simulink model "commhdlQPSKTxRxLoopback"  (R2025b)
settings: Solver=FixedStepDiscrete  StartTime=0.0  StopTime=0.03  RelTol=1e-3
PostLoadFcn:
  | hScopeConfig = get_param([gcs '/Receiver/QPSK Rx/Frequency and Time Synchronizer/Symbol Synchronizer/No HDL/QPSK Receiver Eye Diagram'],'ScopeConfiguration');
  | 
  | hScopeConfig.OpenAtSimulationStart = false;
  | hScopeConfig.Visible = false;
  | SamplesPerSymbol = 4;
  | %UpsamplesRx = 1;
  | clear hScopeConfig
InitFcn:
  | % RxAlign decoder latency (flat_simfix): 41 = netlist value used for HDL; set
  | % rxAlignLat = 25 in the base workspace before a model-level simulation.
  | if ~exist('rxAlignLat','var'), rxAlignLat = uint16(41); end
  | commhdlQPSKTxRxModelInit;
  | % Rate bridge: ADRV9002/Jupiter radio runs at 15.36 MHz = 2x the 7.68 MHz
  | % (4 samples/symbol @ Rsym=1.92 MHz) the QPSK Rx requires. The deployed
  | % Receiver must downsample the ADC stream by 2. UpsamplesRx=1 fed the QPSK
  | % Rx 8 sps (2x-upsampled) and broke symbol sync / the loopback bit check.
  | UpsamplesRx = 1;   %% T8 RATE FIX: rail 15.36e6 == ADC bus rate,
  | %% no ingress decimation (was 2 when the rail sat on the 7.68e6 rung)
  | UpsamplesTx = 1;
  | clear simTimingOffset;
StopFcn:
  | if exist('simTimingOffset','var')
  |   disp('Simulation completed');
  |   %QPSKTxRxVerification;
  | end
undefined symbols (not defined in the file or in its folder): Add, Config, fsym, randsrc, RandStream, Rsym, rxAlignLat, Shift
libraries: hdlsllib x141, simulink x45, dspsigops x30, dsphdlfiltering2 x6, dsphdlsigops2 x4, dsphdlmathfun2 x4, commdigbbndpm3 x4, dspmlti4 x2, commchan3 x1, commrflib2 x1, commcnvcod2 x1
(part 5 of 9)

== system commhdlQPSKTxRxLoopback/Receiver/QPSK Rx/Frequency and Time Synchronizer/Preamble Detector/FIFO ==
  in : Inport
  push : Inport  Port=2
  pop : Inport  Port=3
  reset : Inport  Port=4
  Delay1 : Delay  DelayLength=1
  Pop Counter : hdlsllib/Sources/HDL Counter  CountType=Count limited  CountInit=0  CountStep=1  CountMax=fifoSize -1  CountFromType=Initial value  CountFrom=0  CountResetPort=on  CountLoadPort=off  CountEnbPort=on  CountDirPort=off  CountHitOutputPort=off  CountDataType=Unsigned  CountWordLen=nextpow2(fifoSize)  CountFracLen=0  CountSampTime=1
  Push Counter : hdlsllib/Sources/HDL Counter  CountType=Count limited  CountInit=0  CountStep=1  CountMax=fifoSize -1  CountFromType=Initial value  CountFrom=0  CountResetPort=on  CountLoadPort=off  CountEnbPort=on  CountDirPort=off  CountHitOutputPort=off  CountDataType=Unsigned  CountWordLen=nextpow2(fifoSize)  CountFracLen=0  CountSampTime=1
  Simple Dual Port RAM : hdlsllib/HDL RAMs/Simple Dual Port RAM  ram_size=nextpow2(fifoSize)
  Validate Input Push Pop : Subsystem
  out : Outport
  numEntries : Outport  Port=2
  validPop : Outport  Port=3
  wires:
  Delay1/1 -> Push Counter/1, Pop Counter/1
  in/1 -> Simple Dual Port RAM/1
  reset/1 -> Validate Input Push Pop/1(rst), Delay1/1
  Validate Input Push Pop/2(valid pop) -> Pop Counter/2, validPop/1
  Validate Input Push Pop/1(valid push) -> Push Counter/2, Simple Dual Port RAM/3
  pop/1 -> Validate Input Push Pop/3(pop)
  push/1 -> Validate Input Push Pop/2(push)
  Pop Counter/1 -> Simple Dual Port RAM/4
  Push Counter/1 -> Simple Dual Port RAM/2
  Simple Dual Port RAM/1 -> out/1
  Validate Input Push Pop/3(numEntries) -> numEntries/1

== system commhdlQPSKTxRxLoopback/Receiver/QPSK Rx/Frequency and Time Synchronizer/Preamble Detector/No HDL ==
  In1 : Inport
  In2 : Inport  Port=2
  Enable : EnablePort
  Correlation Time Scope : Scope  NumInputPorts=2
      settings: TimeUnits=Metric (based on Time Span)  Title=Time Plot of Preamble Detection  ActiveDisplayYMinimum=-0.38501295493915666  ActiveDisplayYMaximum=3.4651165944524109  YLabel=Amplitude
  Data Type Conversion : DataTypeConversion  OutDataTypeStr=double  SaturateOnIntegerOverflow=off  RndMeth=Floor
  Data Type Conversion1 : DataTypeConversion  OutDataTypeStr=double  SaturateOnIntegerOverflow=off  RndMeth=Floor
  To Workspace : ToWorkspace  VariableName=simPeakFind  SampleTime=-1
      settings: Save2DSignal=2-D array (concatenate along first dimension)
  wires:
  Data Type Conversion1/1 -> Correlation Time Scope/2  "Threshold"
  In2/1 -> Data Type Conversion1/1
  Data Type Conversion/1 -> To Workspace/1, Correlation Time Scope/1  "Correlation Value"
  In1/1 -> Data Type Conversion/1

== system commhdlQPSKTxRxLoopback/Receiver/QPSK Rx/Frequency and Time Synchronizer/Preamble Detector/Peak Search ==
  note: peak picker
  corr : Inport
  thresholdExceeded : Inport  Port=2
  validIn : Inport  Port=3
  Compare To Constant : simulink/Logic and Bit Operations/Compare To Constant  relop===  const=samplesPerFrame1x - 1  OutDataTypeStr=boolean
  Logical Operator : Logic  IconShape=distinctive  AllPortsSameDT=off  OutDataTypeStr=boolean
  Logical Operator4 : Logic  IconShape=distinctive  AllPortsSameDT=off  OutDataTypeStr=boolean
  Relational Operator : RelationalOperator  Operator=>  OutDataTypeStr=boolean  InputSameDT=off
  Terminator : Terminator
  Unit Delay Enabled Synchronous : hdlsllib/Discrete/Unit Delay Enabled Synchronous  InitialCondition=0.0  SampleTime=-1
  Unit Delay Enabled Synchronous1 : hdlsllib/Discrete/Unit Delay Enabled Synchronous  InitialCondition=0.0  SampleTime=-1
  Unit Delay Enabled Resettable Synchronous : hdlsllib/Discrete/Unit Delay Enabled Resettable Synchronous  InitialCondition=0.0  SampleTime=-1
  Unit Delay Enabled Resettable Synchronous1 : hdlsllib/Discrete/Unit Delay Enabled Resettable Synchronous  InitialCondition=0.0  SampleTime=-1
  timing Reference : hdlsllib/Sources/HDL Counter  CountType=Count limited  CountInit=0  CountStep=1  CountMax=samplesPerFrame1x - 1  CountFromType=Initial value  CountFrom=0  CountResetPort=off  CountLoadPort=off  CountEnbPort=on  CountDirPort=off  CountHitOutputPort=off  CountDataType=Unsigned  CountWordLen=nextpow2(samplesPerFrame1x - 1)  CountFracLen=0  CountSampTime=1
  timing Reference Long : hdlsllib/Sources/HDL Counter  CountType=Free running  CountInit=0  CountStep=1  CountMax=samplesPerFrame1x - 1  CountFromType=Initial value  CountFrom=0  CountResetPort=off  CountLoadPort=off  CountEnbPort=on  CountDirPort=off  CountHitOutputPort=off  CountDataType=Unsigned  CountWordLen=32  CountFracLen=0  CountSampTime=1
  timingOffset : Outport
  done : Outport  Port=2
  success : Outport  Port=3
  wires:
  validIn/1 -> Logical Operator/1, timing Reference/1, timing Reference Long/1
  timing Reference Long/1 -> Unit Delay Enabled Synchronous1/1
  timing Reference/1 -> Unit Delay Enabled Synchronous/1, Compare To Constant/1
  thresholdExceeded/1 -> Unit Delay Enabled Resettable Synchronous1/2, Unit Delay Enabled Resettable Synchronous1/1, Logical Operator4/2
  corr/1 -> Unit Delay Enabled Resettable Synchronous/1, Relational Operator/1
  Compare To Constant/1 -> Logical Operator/2
  Logical Operator/1 -> Unit Delay Enabled Resettable Synchronous1/3, done/1, Unit Delay Enabled Resettable Synchronous/3
  Relational Operator/1 -> Logical Operator4/1
  Unit Delay Enabled Resettable Synchronous/1 -> Relational Operator/2
  Unit Delay Enabled Resettable Synchronous1/1 -> success/1
  Logical Operator4/1 -> Unit Delay Enabled Synchronous/2, Unit Delay Enabled Synchronous1/2, Unit Delay Enabled Resettable Synchronous/2
  Unit Delay Enabled Synchronous/1 -> timingOffset/1
  Unit Delay Enabled Synchronous1/1 -> Terminator/1

== system commhdlQPSKTxRxLoopback/Receiver/QPSK Rx/Frequency and Time Synchronizer/Preamble Detector/Timing Adjust ==
  timingOffset : Inport
  timingOffsetValid : Inport  Port=2
  dataIn : Inport  Port=3
  validIn : Inport  Port=4
  Delay{,1..4} (5 alike) : Delay  DelayLength=1
  Logical Operator : Logic  AllPortsSameDT=off  OutDataTypeStr=boolean
  Logical Operator1 : Logic  Operator=NOT  AllPortsSameDT=off  OutDataTypeStr=boolean
  Logical Operator2 : Logic  Inputs=3  AllPortsSameDT=off  OutDataTypeStr=boolean
  No HDL : Subsystem
  Relational Operator : RelationalOperator  Operator===  OutDataTypeStr=boolean  InputSameDT=off
  State Register : hdlsllib/Discrete/Unit Delay Enabled Resettable Synchronous  InitialCondition=0.0  SampleTime=-1
  Unit Delay Enabled Synchronous3 : hdlsllib/Discrete/Unit Delay Enabled Synchronous  InitialCondition=0.0  SampleTime=-1
  timing Reference : hdlsllib/Sources/HDL Counter  CountType=Count limited  CountInit=0  CountStep=1  CountMax=searchSamples - 1  CountFromType=Initial value  CountFrom=0  CountResetPort=off  CountLoadPort=off  CountEnbPort=on  CountDirPort=off  CountHitOutputPort=off  CountDataType=Unsigned  CountWordLen=nextpow2(searchSamples - 1)  CountFracLen=0  CountSampTime=1
  dataOut : Outport
  validOut : Outport  Port=2
  SyncPulse : Outport  Port=3
  wires:
  Delay4/1 -> dataOut/1
  Delay3/1 -> validOut/1
  timingOffset/1 -> Unit Delay Enabled Synchronous3/1
  Unit Delay Enabled Synchronous3/1 -> Relational Operator/2
  Delay/1 -> SyncPulse/1
  validIn/1 -> timing Reference/1, Logical Operator2/1, No HDL/1(validIn), Delay3/1
  State Register/1 -> Logical Operator2/3, Delay1/1
  Logical Operator1/1 -> Logical Operator/2
  Relational Operator/1 -> Logical Operator2/2
  Logical Operator2/1 -> No HDL/3(syncPulse), Delay/1, Delay2/1
  Delay2/1 -> State Register/3
  Logical Operator/1 -> State Register/1, State Register/2, Unit Delay Enabled Synchronous3/2
  timing Reference/1 -> No HDL/2(timingOffset), Relational Operator/1
  timingOffsetValid/1 -> Logical Operator/1
  Delay1/1 -> Logical Operator1/1
  dataIn/1 -> Delay4/1

== system commhdlQPSKTxRxLoopback/Receiver/QPSK Rx/Frequency and Time Synchronizer/Symbol Synchronizer/Gardner TED ==
  data : Inport
  strobe : Inport  Port=2
  Constant : Constant  Value=0  OutDataTypeStr=Inherit: Inherit via back propagation  SampleTime=1/(Rsym*SamplesPerSymbol)
  Delay10 : Delay  DelayLength=4
  GTED : Subsystem
  Switch : Switch  Criteria=u2 ~= 0  InputSameDT=off
  e : Outport  VectorParamsAs1DForOutWhenUnconnected=off
  wires:
  Constant/1 -> Switch/3
  Switch/1 -> e/1
  strobe/1 -> Delay10/1
  data/1 -> GTED/1(In1)
  GTED/1(Out1) -> Switch/1
  Delay10/1 -> Switch/2

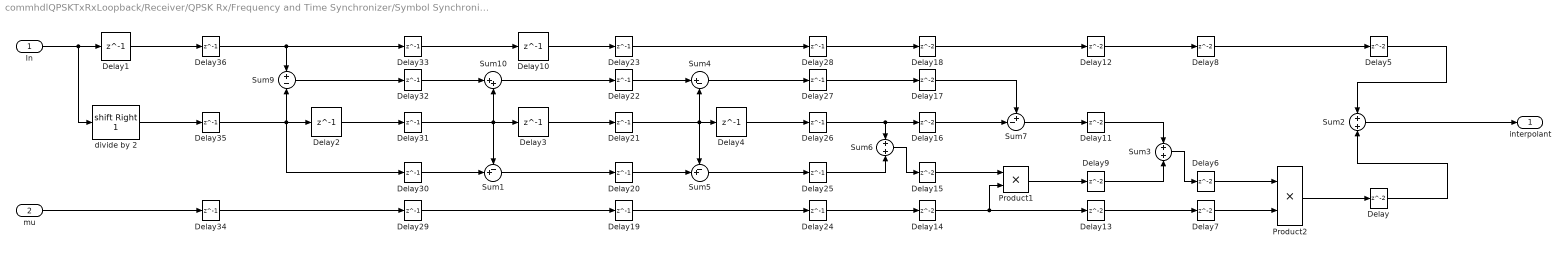
== system commhdlQPSKTxRxLoopback/Receiver/QPSK Rx/Frequency and Time Synchronizer/Symbol Synchronizer/Interpolation Filter ==
  In : Inport
  mu : Inport  Port=2
  Delay{,5..9,11..18} (14 alike) : Delay
  Delay{1..4,10} (5 alike) : Delay  DelayLength=1  InitialCondition=0
  Delay{19..36} (18 alike) : Delay  DelayLength=1
  Product1 : Product  OutDataTypeStr=fixdt(1,16,10)  RndMeth=Zero
  Product2 : Product  RndMeth=Zero  OutDataTypeStr=Inherit: Same as first input
  Sum1 : Sum  Inputs=-+|
  Sum10 : Sum  Inputs=|++
  Sum2 : Sum  Inputs=+|+
  Sum3 : Sum  Inputs=+|+  OutDataTypeStr=fixdt(1,16,10)
  Sum4 : Sum  Inputs=|+-
  Sum5 : Sum  Inputs=-+|
  Sum6 : Sum  Inputs=+|+  OutDataTypeStr=fixdt(1,16,11)  SaturateOnIntegerOverflow=on
  Sum7 : Sum  Inputs=+-|  OutDataTypeStr=fixdt(1,16,10)
  Sum9 : Sum  Inputs=+-
  divide by 2 : ArithShift  BitShiftNumber=1  BitShiftDirection=Right
  interpolant : Outport
  wires:
  Sum9/1 -> Delay32/1
  In/1 -> divide by 2/1, Delay1/1
  Sum2/1 -> interpolant/1
  Sum7/1 -> Delay11/1
  Product1/1 -> Delay9/1
  Product2/1 -> Delay/1
  Sum3/1 -> Delay6/1
  Sum1/1 -> Delay20/1
  Delay3/1 -> Delay21/1
  Sum10/1 -> Delay22/1
  Delay2/1 -> Delay31/1
  Delay1/1 -> Delay36/1
  divide by 2/1 -> Delay35/1
  Delay/1 -> Sum2/2
  Delay5/1 -> Sum2/1
  Delay6/1 -> Product2/1
  Delay7/1 -> Product2/2
  Delay8/1 -> Delay5/1
  Delay9/1 -> Sum3/2
  Delay11/1 -> Sum3/1
  Delay12/1 -> Delay8/1
  Delay13/1 -> Delay7/1
  Delay14/1 -> Delay13/1, Product1/2
  Delay15/1 -> Product1/1
  Delay16/1 -> Sum7/2
  Delay17/1 -> Sum7/1
  Delay18/1 -> Delay12/1
  mu/1 -> Delay34/1
  Sum5/1 -> Delay25/1
  Delay4/1 -> Delay26/1
  Sum4/1 -> Delay27/1
  Delay10/1 -> Delay23/1
  Delay24/1 -> Delay14/1
  Sum6/1 -> Delay15/1
  Delay26/1 -> Delay16/1, Sum6/1
  Delay27/1 -> Delay17/1
  Delay28/1 -> Delay18/1
  Delay25/1 -> Sum6/2
  Delay19/1 -> Delay24/1
  Delay20/1 -> Sum5/2
  Delay21/1 -> Sum4/2, Sum5/1, Delay4/1
  Delay22/1 -> Sum4/1
  Delay23/1 -> Delay28/1
  Delay29/1 -> Delay19/1
  Delay30/1 -> Sum1/2
  Delay31/1 -> Sum1/1, Sum10/2, Delay3/1
  Delay32/1 -> Sum10/1
  Delay33/1 -> Delay10/1
  Delay34/1 -> Delay29/1
  Delay35/1 -> Delay30/1, Delay2/1, Sum9/2
  Delay36/1 -> Delay33/1, Sum9/1

== system commhdlQPSKTxRxLoopback/Receiver/QPSK Rx/Frequency and Time Synchronizer/Symbol Synchronizer/Loop Filter ==
  note: Proportional-Plus-Integrator Loop Filter,
      | Infinite DC Response to guarantee convergence
  e : Inport
  Add : Sum
  Add2 : Sum  Inputs=|++  OutDataTypeStr=Inherit: Same as first input
  Data Type Conversion17 : DataTypeConversion  OutDataTypeStr=fixdt(1,11,10)  RndMeth=Floor
  Delay : Delay  DelayLength=1
  Delay1 : Delay  DelayLength=1  InitialCondition=0
  Delay2 : Delay  InitialCondition=0
  Delay3 : Delay  InitialCondition=0
  Delay4 : Delay  DelayLength=1  InitialCondition=0
  Delay5 : Delay  InitialCondition=0
  Delay6 : Delay  DelayLength=1
  IntegClamp : Saturate  UpperLimit=0.06  LowerLimit=-0.06
  K1 : Gain  Gain=fi(SSLoopFilterPropGain,1,24,24)  ParamDataTypeStr=Inherit: Inherit from 'Gain'  OutDataTypeStr=fixdt(1,30,23)
  K2 : Gain  Gain=fi(SSLoopFilterIntegGain,1,24,24)  ParamDataTypeStr=Inherit: Inherit from 'Gain'  OutDataTypeStr=fixdt(1,30,23)
  v : Outport
  wires:
  Delay/1 -> Add2/2
  Delay5/1 -> Delay6/1
  Delay3/1 -> Delay1/1
  e/1 -> Delay2/1
  Add/1 -> Data Type Conversion17/1
  Delay1/1 -> Add/1
  Delay4/1 -> Add/2
  Delay2/1 -> K1/1, K2/1
  Data Type Conversion17/1 -> v/1
  K2/1 -> Delay5/1
  K1/1 -> Delay3/1
  Delay6/1 -> Add2/1
  Add2/1 -> IntegClamp/1
  IntegClamp/1 -> Delay/1, Delay4/1

== system commhdlQPSKTxRxLoopback/Receiver/QPSK Rx/Frequency and Time Synchronizer/Symbol Synchronizer/No HDL ==
  data : Inport
  valid : Inport  Port=2
  Data Type Conversion : DataTypeConversion  OutDataTypeStr=double  SaturateOnIntegerOverflow=off  RndMeth=Floor
  No HDL : Subsystem
  QPSK Receiver Eye Diagram : EyeDiagramBlock  WindowPosition=[403.000000,370.000000,417.000000,506.000000,]  ScopeFrameLocation=window  SamplesPerSymbol=SamplesPerSymbol  SymbolsPerTrace=1  Title=RRC Matched Filtered Output  YLimits=[-1.1602,1.2629]
      settings: OpenAtSimulationStart=off
  Unit Delay Enabled Synchronous : hdlsllib/Discrete/Unit Delay Enabled Synchronous  InitialCondition=0.0  SampleTime=-1
  wires:
  data/1 -> No HDL/1(data), Unit Delay Enabled Synchronous/1
  Unit Delay Enabled Synchronous/1 -> Data Type Conversion/1
  valid/1 -> Unit Delay Enabled Synchronous/2, No HDL/Enable
  Data Type Conversion/1 -> QPSK Receiver Eye Diagram/1

== system commhdlQPSKTxRxLoopback/Receiver/QPSK Rx/Frequency and Time Synchronizer/Symbol Synchronizer/Rate Handle ==
  dataIn : Inport
  strobe : Inport  Port=2
  validIn : Inport  Port=3
  Compare To Constant : simulink/Logic and Bit Operations/Compare To Constant  relop===  const=0  OutDataTypeStr=boolean
  Constant : Constant  Value=false  SampleTime=-1
  FIFO : Subsystem  mask{fifoSize=32, pushFullDiag=Error, popEmptyDiag=Ignore}
      mask prompts: fifoSize "FIFO size:"; pushFullDiag "Push full FIFO:"; popEmptyDiag "Pop empty FIFO:"
      mask TypeOptions pushFullDiag: Ignore | Warning | Error
      mask TypeOptions popEmptyDiag: Ignore | Warning | Error
  HDL Counter : hdlsllib/Sources/HDL Counter  CountType=Count limited  CountInit=0  CountStep=1  CountMax=SamplesPerSymbol - 1  CountFromType=Initial value  CountFrom=0  CountResetPort=off  CountLoadPort=off  CountEnbPort=on  CountDirPort=off  CountHitOutputPort=off  CountDataType=Unsigned  CountWordLen=max(1, nextpow2(SamplesPerSymbol - 1))  CountFracLen=0  CountSampTime=1
  Logical Operator : Logic  AllPortsSameDT=off  OutDataTypeStr=boolean
  Terminator : Terminator
  dataOut : Outport
  validOut : Outport  Port=2
  wires:
  strobe/1 -> FIFO/2(push)
  dataIn/1 -> FIFO/1(in)
  validIn/1 -> Logical Operator/1, HDL Counter/1
  HDL Counter/1 -> Compare To Constant/1
  Compare To Constant/1 -> Logical Operator/2
  Logical Operator/1 -> FIFO/3(pop)
  FIFO/1(out) -> dataOut/1
  FIFO/3(validPop) -> validOut/1
  FIFO/2(numEntries) -> Terminator/1
  Constant/1 -> FIFO/4(reset)

== system commhdlQPSKTxRxLoopback/Transmitter/QPSK Tx/Bit Packetizer/Data Bits FIFO/No HDL ==
  push : Inport
  pop : Inport  Port=2
  MATLAB Function : MATLAB Function  TreatAsAtomicUnit=on
  No HDL : Subsystem
  wires:
  push/1 -> MATLAB Function/1(wr), No HDL/1(push)
  pop/1 -> MATLAB Function/2(rd), No HDL/5(pop)
  MATLAB Function/2(ncount) -> No HDL/3(ncount)
  MATLAB Function/1(full) -> No HDL/2(full)
  MATLAB Function/3(empty) -> No HDL/4(empty)

== system commhdlQPSKTxRxLoopback/Transmitter/QPSK Tx/Bit Packetizer/Preamble Bits Generator/Preamble Bits Store ==
  note: The Preamble is padded with zeros in the LUT such that
      | the length is the 2^nextpow2(length(Preamble)) for
      | efficient resource mapping to RAM
  actualPreamble : Inport
  sampleCount : Inport  Port=2
  Constant : Constant  OutDataTypeStr=boolean  SampleTime=1/(Rsym*SamplesPerSymbol)
  Extract Bits : simulink/Logic and Bit Operations/Extract Bits  bitsToExtract=Range of bits  numBits=8  bitIdxRange=[0 nextpow2(length(Preamble))-1]  outScalingMode=Treat bit field as an integer
  Preamble : LookupNDDirect  NumberOfTableDimensions=1  Table=[Preamble;false(32-length(Preamble),1)]  DiagnosticForOutOfRangeInput=Error
  Switch : Switch  Criteria=u2 ~= 0  Threshold=1  SaturateOnIntegerOverflow=off  InputSameDT=off
  preamble : Outport
  wires:
  Switch/1 -> preamble/1
  Constant/1 -> Switch/3
  Extract Bits/1 -> Preamble/1
  Preamble/1 -> Switch/1
  sampleCount/1 -> Extract Bits/1
  actualPreamble/1 -> Switch/2

== system commhdlQPSKTxRxLoopback/TxRxComposite/Receiver/QPSK Rx/Automatic Gain Control/Error Detector ==
  dataIn : Inport
  Add1 : Sum  Inputs=+-
  Conj : Math  Operator=conj
  Data Type Duplicate : DataTypeDuplicate
  Delay{,1..3} (4 alike) : Delay
  Product : Product
  Ref : Constant  Value=Ref  OutDataTypeStr=Inherit: Inherit via back propagation  SampleTime=-1
  err : Outport
  wires:
  Add1/1 -> Delay3/1
  Delay2/1 -> Add1/2
  Product/1 -> Delay2/1
  Delay/1 -> Product/2
  Delay3/1 -> err/1
  Delay1/1 -> Product/1
  Conj/1 -> Delay/1
  dataIn/1 -> Conj/1, Data Type Duplicate/2, Delay1/1
  Ref/1 -> Data Type Duplicate/1, Add1/1

== system commhdlQPSKTxRxLoopback/TxRxComposite/Receiver/QPSK Rx/Automatic Gain Control/Loop Filter ==
  note: Fixed point precision loss warnings
      | are supressed in Mask Init Callback
  err : Inport
  agc_loop_gain : Inport  Port=2  OutDataTypeStr=uint32  SampleTime=1/(Rsym*SamplesPerSymbol)
  Add : Sum  Inputs=|++  OutDataTypeStr=Inherit: Same as first input
  Delay1 : Delay  DelayLength=1
  Delay2 : Delay
  Delay3 : Delay
  Gain1 : Gain  Gain=LFG  OutDataTypeStr=fixdt(1,34,28)
      mask init:
      | Simulink.suppressDiagnostic(gcb, 'SimulinkFixedPoint:util:fxpParameterPrecisionLoss');
  LGMux_agc_loop_gain : MATLAB Function  TreatAsAtomicUnit=on
  LGProd_agc_loop_gain : Product  OutDataTypeStr=fixdt(1,34,28)
  LGSw_agc_loop_gain : Switch  Criteria=u2 ~= 0  OutDataTypeStr=fixdt(1,34,28)
  gain : Outport
  wires:
  LGSw_agc_loop_gain/1 -> Delay2/1
  LGProd_agc_loop_gain/1 -> LGSw_agc_loop_gain/1
  Delay1/1 -> gain/1, Add/2
  Delay3/1 -> LGProd_agc_loop_gain/1, Gain1/1
  Gain1/1 -> LGSw_agc_loop_gain/3
  LGMux_agc_loop_gain/2(nz) -> LGSw_agc_loop_gain/2
  err/1 -> Delay3/1
  Add/1 -> Delay1/1
  Delay2/1 -> Add/1
  LGMux_agc_loop_gain/1(coeff) -> LGProd_agc_loop_gain/2
  agc_loop_gain/1 -> LGMux_agc_loop_gain/1(axi)

== system commhdlQPSKTxRxLoopback/TxRxComposite/Receiver/QPSK Rx/FEC Decoder Wrapper/VitGate ==
  pairIn : Inport
  rstIn : Inport  Port=2
  Enable : EnablePort
  Viterbi : commcnvcod2/Viterbi Decoder  trellis=poly2trellis(5, [35 23])  isPunctured=off  punctureVector=[1; 1; 0; 1; 0; 1]  erasures=off  dectype=Hard decision  nsdecb=4  runSigValErrCheck=off  tbdepth=25  opmode=Continuous  reset=on  delayedResetAction=on  smWordLength=16  outDataType=boolean
  decOut : Outport
  wires:
  Viterbi/1 -> decOut/1
  rstIn/1 -> Viterbi/2
  pairIn/1 -> Viterbi/1

== system commhdlQPSKTxRxLoopback/TxRxComposite/Receiver/QPSK Rx/Frequency and Time Synchronizer/Carrier Synchronizer ==
  dataIn : Inport
  internalRst : Inport  Port=2
  validIn : Inport  Port=3
  manualRst : Inport  Port=4
  cs_prop_gain : Inport  Port=5  OutDataTypeStr=uint32  SampleTime=1/(Rsym*SamplesPerSymbol)
  cs_integ_gain : Inport  Port=6  OutDataTypeStr=uint32  SampleTime=1/(Rsym*SamplesPerSymbol)
  Data Type Conversion2 : DataTypeConversion  OutDataTypeStr=fixdt(1,16,14)  SaturateOnIntegerOverflow=off  RndMeth=Floor
  Delay{,2,5,7,11} (5 alike) : Delay  DelayLength=1
  Delay{1,10,14..15} (4 alike) : Delay  DelayLength=6
  Delay{3..4,6,8..9,12..13} (7 alike) : Delay
  Direct Digital Synthesis : Subsystem
  Logical Operator : Logic  AllPortsSameDT=off  OutDataTypeStr=boolean
  Loop Filter : Subsystem
  Math Function : Math  Operator=conj  SignedPower=on  RndMeth=Zero
  Phase Error Detector : Subsystem
  Product : Product
  dataOut : Outport
  validOut : Outport  Port=2
  wires:
  Delay5/1 -> dataOut/1
  Delay/1 -> Phase Error Detector/1(dataIn)
  Delay1/1 -> Loop Filter/2(validIn)
  Math Function/1 -> Delay3/1
  Data Type Conversion2/1 -> Delay5/1, Delay/1
  Loop Filter/3(rst) -> Logical Operator/2
  Loop Filter/2(valid) -> Direct Digital Synthesis/2(validIn)
  Delay3/1 -> Product/2
  Loop Filter/1(v) -> Direct Digital Synthesis/3(phaseInc)
  cs_integ_gain/1 -> Loop Filter/6(cs_integ_gain)
  cs_prop_gain/1 -> Loop Filter/5(cs_prop_gain)
  Delay12/1 -> Delay11/1
  internalRst/1 -> Delay13/1
  Delay2/1 -> Delay1/1
  Delay13/1 -> Delay12/1
  manualRst/1 -> Loop Filter/4(externalRst), Logical Operator/1
  Delay14/1 -> Delay9/1
  Delay4/1 -> Product/1
  Delay15/1 -> Loop Filter/3(internalRst)
  Delay9/1 -> Delay8/1
  Logical Operator/1 -> Direct Digital Synthesis/1(rst)
  validIn/1 -> Delay14/1
  Product/1 -> Delay6/1
  Delay8/1 -> Delay7/1, Delay2/1
  dataIn/1 -> Delay10/1
  Direct Digital Synthesis/1(expOut) -> Math Function/1
  Delay7/1 -> validOut/1
  Delay6/1 -> Data Type Conversion2/1
  Delay11/1 -> Delay15/1
  Delay10/1 -> Delay4/1
  Phase Error Detector/1(PhaseError) -> Loop Filter/1(e)

== system commhdlQPSKTxRxLoopback/TxRxComposite/Receiver/QPSK Rx/Frequency and Time Synchronizer/Coarse Frequency Compensator ==
  dataIn : Inport
  validIn : Inport  Port=2
  cfo_threshold : Inport  Port=3  OutDataTypeStr=uint32  SampleTime=1/(Rsym*SamplesPerSymbol)
  CFO step change detector : Subsystem
  Coarse Frequency Estimator : Subsystem
  Data Type Conversion2 : DataTypeConversion  OutDataTypeStr=fixdt(1,16,12)  SaturateOnIntegerOverflow=off  RndMeth=Floor
  Data Type Conversion3 : DataTypeConversion  OutDataTypeStr=fixdt(1,21,21)  SaturateOnIntegerOverflow=off  RndMeth=Floor
  Data Type Conversion4 : DataTypeConversion  OutDataTypeStr=fixdt(1,21,0)  ConvertRealWorld=Stored Integer (SI)  SaturateOnIntegerOverflow=off  RndMeth=Floor
  Delay1 : Delay  DelayLength=9
  Delay{11..17} (7 alike) : Delay
  Delay2 : Delay  DelayLength=9
  Delay3 : Delay  DelayLength=6
  Delay4 : Delay  DelayLength=6
  Delay5 : Delay  DelayLength=1
  Delay6 : Delay  DelayLength=1
  Delay7 : Delay  DelayLength=12
  Delay8 : Delay  DelayLength=12
  Gain : Gain  Gain=1/4  ParamDataTypeStr=fixdt(0,2,2)  OutDataTypeStr=Inherit: Same as input
  Math Function : Math  Operator=conj
  NCO : dsphdlsigops2/NCO  PhaseIncrementSource=Input port  PhaseIncrement=100  PhaseOffsetSource=Property  PhaseOffset=0  DitherSource=None  NumDitherBits=4  SamplesPerFrame=1  LUTCompress=off  ResetAction=off  Waveform=Complex exponential  PhasePort=off  SimulateUsing=Code generation  AccumulatorWL=21  PhaseQuantization=on  NumQuantizerAccumulatorBits=14  OutputDataType=Binary point scaling  OutputWL=16  OutputFL=14
  Product1 : Product  OutDataTypeStr=Inherit: Same as first input
  Raise Power to 4 : Subsystem
  Terminator : Terminator
  dataOut : Outport
  rstCS : Outport  Port=2
  validOut : Outport  Port=3
  normalizedFreqEst : Outport  Port=4
  wires:
  Delay8/1 -> Delay4/1, NCO/2
  Raise Power to 4/2(validOut) -> Coarse Frequency Estimator/2(validIn)
  Coarse Frequency Estimator/1(normFreqEst) -> Gain/1
  Delay2/1 -> Delay8/1
  cfo_threshold/1 -> CFO step change detector/2(cfo_threshold)
  Delay16/1 -> Delay17/1
  Delay6/1 -> Raise Power to 4/2(validIn), Delay2/1
  Delay3/1 -> Delay11/1
  Data Type Conversion2/1 -> Raise Power to 4/1(dataIn)
  Delay5/1 -> Data Type Conversion2/1, Delay1/1
  Raise Power to 4/1(dataOut) -> Coarse Frequency Estimator/1(dataIn)
  Delay7/1 -> Delay3/1
  Data Type Conversion4/1 -> NCO/1
  Delay1/1 -> Delay7/1
  Delay13/1 -> dataOut/1
  Product1/1 -> Delay13/1
  validIn/1 -> Delay6/1
  dataIn/1 -> Delay5/1
  Gain/1 -> Data Type Conversion3/1
  Delay4/1 -> Delay14/1
  Delay15/1 -> validOut/1
  Data Type Conversion3/1 -> normalizedFreqEst/1, CFO step change detector/1(In1), Data Type Conversion4/1
  CFO step change detector/1(Out1) -> Delay16/1
  NCO/1 -> Math Function/1
  NCO/2 -> Terminator/1
  Math Function/1 -> Delay12/1
  Delay17/1 -> rstCS/1
  Delay11/1 -> Product1/1
  Delay14/1 -> Delay15/1
  Delay12/1 -> Product1/2

== system commhdlQPSKTxRxLoopback/TxRxComposite/Receiver/QPSK Rx/Frequency and Time Synchronizer/No HDL ==
  In1 : Inport
  In2 : Inport  Port=2
  In3 : Inport  Port=3
  In4 : Inport  Port=4
  Data Type Conversion : DataTypeConversion  OutDataTypeStr=double  SaturateOnIntegerOverflow=off  RndMeth=Floor
  Data Type Conversion1 : DataTypeConversion  OutDataTypeStr=double  SaturateOnIntegerOverflow=off  RndMeth=Floor
  Subsystem : Subsystem
  Unit Delay Enabled Synchronous : hdlsllib/Discrete/Unit Delay Enabled Synchronous  InitialCondition=0.0  SampleTime=-1
  Unit Delay Enabled Synchronous1 : hdlsllib/Discrete/Unit Delay Enabled Synchronous  InitialCondition=0.0  SampleTime=-1
  wires:
  Data Type Conversion/1 -> Unit Delay Enabled Synchronous1/1, Subsystem/1(In1)
  In4/1 -> Unit Delay Enabled Synchronous1/2, Subsystem/Enable
  In2/1 -> Unit Delay Enabled Synchronous/2
  Data Type Conversion1/1 -> Unit Delay Enabled Synchronous/1
  In3/1 -> Data Type Conversion/1
  In1/1 -> Data Type Conversion1/1

== system commhdlQPSKTxRxLoopback/TxRxComposite/Receiver/QPSK Rx/Frequency and Time Synchronizer/Packet Controller ==
  dataIn : Inport
  syncPulse : Inport  Port=2
  validIn : Inport  Port=3
  Delay : Delay  DelayLength=4
  Delay1 : Delay  DelayLength=4
  Delay2 : Delay  DelayLength=4
  End Generator : Subsystem
  Logical Operator : Logic  IconShape=distinctive  AllPortsSameDT=off  OutDataTypeStr=boolean
  MATLAB Function : MATLAB Function  TreatAsAtomicUnit=on
  Time Scope End Generator : Scope  Commented=on  NumInputPorts=2
      settings: SampleTime=1  ActiveDisplayYMinimum=-0.048155737704917989  ActiveDisplayYMaximum=1.0464480874316939  YLabel=Amplitude  DataLoggingVariableName=ScopeData2
  sample discard controller : MATLAB Function  TreatAsAtomicUnit=on
  dataOut : Outport
  startOut : Outport  Port=2
  endOut : Outport  Port=3
  validOut : Outport  Port=4
  wires:
  sample discard controller/4(validOut) -> validOut/1
  Delay/1 -> sample discard controller/1(dataIn)
  sample discard controller/2(startOut) -> startOut/1
  End Generator/1(endOut) -> sample discard controller/4(endIn), Time Scope End Generator/1
  Logical Operator/1 -> Delay2/1, End Generator/2(rst), Time Scope End Generator/2
  Delay1/1 -> End Generator/1(validIn), sample discard controller/2(validIn)
  dataIn/1 -> Delay/1
  sample discard controller/1(dataOut) -> dataOut/1
  MATLAB Function/1(out) -> Logical Operator/2
  sample discard controller/3(endOut) -> endOut/1
  syncPulse/1 -> MATLAB Function/2(syncPulse)
  Delay2/1 -> sample discard controller/3(startIn)
  validIn/1 -> MATLAB Function/1(valid), Delay1/1, Logical Operator/1

== system commhdlQPSKTxRxLoopback/TxRxComposite/Receiver/QPSK Rx/Frequency and Time Synchronizer/Phase Ambiguity Estimation and Correction ==
  dataIn : Inport
  syncPulseIn : Inport  Port=2
  validIn : Inport  Port=3
  Average Estimates : Subsystem
  Delay : Delay  DelayLength=32
  Delay1 : Delay  DelayLength=32
  Delay10 : Delay  DelayLength=15 + 7
  Delay11 : Delay  DelayLength=5
  Delay12 : Delay  DelayLength=5
  Delay13 : Delay  DelayLength=5
  Delay2 : Delay  DelayLength=32
  Delay3 : Delay  DelayLength=8
  Delay4 : Delay  DelayLength=8
  Delay5 : Delay  DelayLength=8
  Delay6 : Delay  DelayLength=1
  Delay7 : Delay  DelayLength=1
  Delay8 : Delay  DelayLength=1
  Delay9 : Delay  DelayLength=10
  EstDataLookback : Delay  DelayLength=6
  EstVldLookback : Delay  DelayLength=6
  Phase Ambiguity Corrector : Subsystem
  Phase Ambiguity Estimator : Subsystem
  dataOut : Outport
  syncPulseOut : Outport  Port=2
  validOut : Outport  Port=3
  wires:
  Delay9/1 -> syncPulseOut/1
  Phase Ambiguity Corrector/2(validOut) -> validOut/1
  Phase Ambiguity Corrector/1(dataOut) -> dataOut/1
  Delay6/1 -> Delay10/1
  Average Estimates/1(avgEst) -> Phase Ambiguity Corrector/2(estimate)
  Delay8/1 -> Phase Ambiguity Corrector/1(dataIn)
  Delay3/1 -> Delay1/1
  Delay7/1 -> Phase Ambiguity Corrector/3(validIn)
  Delay/1 -> EstDataLookback/1, Delay13/1
  Delay1/1 -> Delay11/1
  Phase Ambiguity Estimator/3(validOut) -> Average Estimates/3(validIn)
  validIn/1 -> Delay4/1
  Delay4/1 -> Delay2/1
  Delay2/1 -> EstVldLookback/1, Delay12/1
  syncPulseIn/1 -> Phase Ambiguity Estimator/2(syncPulse), Delay3/1
  Delay12/1 -> Delay7/1
  Delay11/1 -> Delay6/1
  Delay13/1 -> Delay8/1
  EstDataLookback/1 -> Phase Ambiguity Estimator/1(dataIn)
  dataIn/1 -> Delay5/1
  Delay5/1 -> Delay/1
  EstVldLookback/1 -> Phase Ambiguity Estimator/3(validIn)
  Phase Ambiguity Estimator/1(endOut) -> Average Estimates/1(endIn)
  Delay10/1 -> Delay9/1
  Phase Ambiguity Estimator/2(estOut) -> Average Estimates/2(estin)

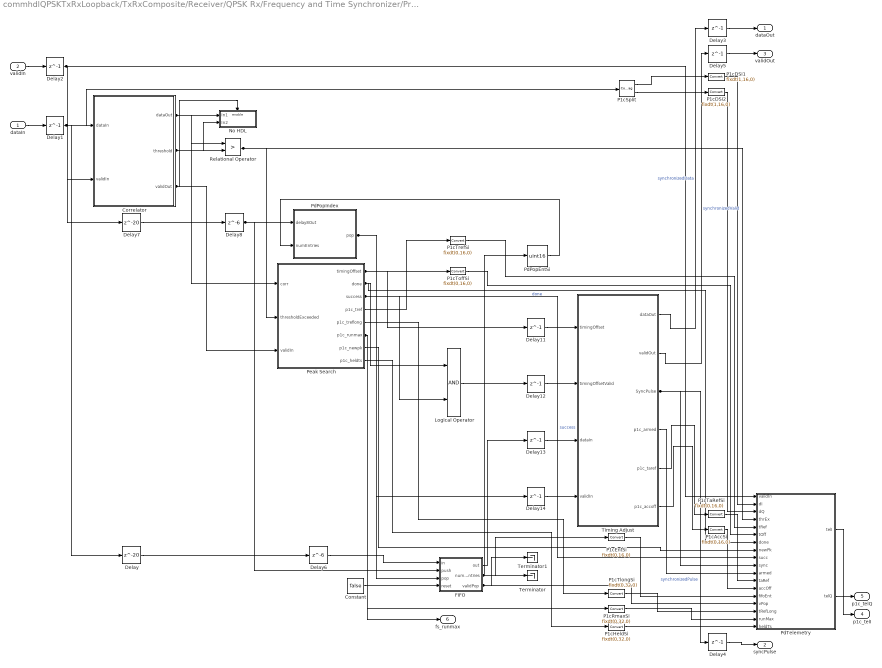
== system commhdlQPSKTxRxLoopback/TxRxComposite/Receiver/QPSK Rx/Frequency and Time Synchronizer/Preamble Detector ==
  dataIn : Inport
  validIn : Inport  Port=2
  Constant : Constant  Value=false  SampleTime=-1
  Correlator : Subsystem
  Delay : Delay  DelayLength=20
  Delay{1..5,11..14} (9 alike) : Delay  DelayLength=1
  Delay6 : Delay  DelayLength=6
  Delay7 : Delay  DelayLength=20
  Delay8 : Delay  DelayLength=6
  FIFO : Subsystem  mask{fifoSize=searchSamples, pushFullDiag=Error, popEmptyDiag=Error}
      mask prompts: fifoSize "FIFO size:"; pushFullDiag "Push full FIFO:"; popEmptyDiag "Pop empty FIFO:"
      mask TypeOptions pushFullDiag: Ignore | Warning | Error
      mask TypeOptions popEmptyDiag: Ignore | Warning | Error
  Logical Operator : Logic  AllPortsSameDT=off  OutDataTypeStr=boolean
  No HDL : Subsystem
  P1cAccSi : DataTypeConversion  OutDataTypeStr=fixdt(0,16,0)  ConvertRealWorld=Stored Integer (SI)  SaturateOnIntegerOverflow=off  RndMeth=Floor
  P1cDSi1 : DataTypeConversion  OutDataTypeStr=fixdt(1,16,0)  ConvertRealWorld=Stored Integer (SI)  SaturateOnIntegerOverflow=off  RndMeth=Floor
  P1cDSi2 : DataTypeConversion  OutDataTypeStr=fixdt(1,16,0)  ConvertRealWorld=Stored Integer (SI)  SaturateOnIntegerOverflow=off  RndMeth=Floor
  P1cEntSi : DataTypeConversion  OutDataTypeStr=fixdt(0,16,0)  ConvertRealWorld=Stored Integer (SI)  SaturateOnIntegerOverflow=off  RndMeth=Floor
  P1cHeldSi : DataTypeConversion  OutDataTypeStr=fixdt(0,32,0)  ConvertRealWorld=Stored Integer (SI)  SaturateOnIntegerOverflow=off  RndMeth=Floor
  P1cRmaxSi : DataTypeConversion  OutDataTypeStr=fixdt(0,32,0)  ConvertRealWorld=Stored Integer (SI)  SaturateOnIntegerOverflow=off  RndMeth=Floor
  P1cSplit : ComplexToRealImag
  P1cTaRefSi : DataTypeConversion  OutDataTypeStr=fixdt(0,16,0)  ConvertRealWorld=Stored Integer (SI)  SaturateOnIntegerOverflow=off  RndMeth=Floor
  P1cTlongSi : DataTypeConversion  OutDataTypeStr=fixdt(0,32,0)  ConvertRealWorld=Stored Integer (SI)  SaturateOnIntegerOverflow=off  RndMeth=Floor
  P1cToffSi : DataTypeConversion  OutDataTypeStr=fixdt(0,16,0)  ConvertRealWorld=Stored Integer (SI)  SaturateOnIntegerOverflow=off  RndMeth=Floor
  P1cTrefSi : DataTypeConversion  OutDataTypeStr=fixdt(0,16,0)  ConvertRealWorld=Stored Integer (SI)  SaturateOnIntegerOverflow=off  RndMeth=Floor
  PdPopEntSi : DataTypeConversion  OutDataTypeStr=uint16  ConvertRealWorld=Stored Integer (SI)  SaturateOnIntegerOverflow=off  RndMeth=Floor
  PdPopIndex : MATLAB Function  TreatAsAtomicUnit=on
  PdTelemetry : MATLAB Function  TreatAsAtomicUnit=on
  Peak Search : Subsystem  VariantControl=new  mask{samplesPerFrame=searchSamples}
      mask prompts: samplesPerFrame "Number of samples to search:"
      mask init:
      | samplesPerFrame1x            = samplesPerFrame;
      |     searchDuration               = samplesPerFrame1x;
  Relational Operator : RelationalOperator  Operator=>  OutDataTypeStr=boolean  InputSameDT=off
  Terminator : Terminator
  Terminator1 : Terminator
  Timing Adjust : Subsystem
  dataOut : Outport
  syncPulse : Outport  Port=2
  validOut : Outport  Port=3
  p1c_telI : Outport  Port=4
  p1c_telQ : Outport  Port=5
  fs_runmax : Outport  Port=6
  wires:
  PdTelemetry/1(telI) -> p1c_telI/1
  P1cAccSi/1 -> PdTelemetry/13(accOff)
  P1cTaRefSi/1 -> PdTelemetry/12(taRef)
  P1cDSi1/1 -> PdTelemetry/2(dI)
  Delay4/1 -> syncPulse/1
  P1cHeldSi/1 -> PdTelemetry/18(heldTs)
  P1cRmaxSi/1 -> PdTelemetry/17(runMax)
  P1cEntSi/1 -> PdTelemetry/14(fifoEnt)
  Timing Adjust/6(p1c_accoff) -> P1cAccSi/1
  Timing Adjust/5(p1c_taref) -> P1cTaRefSi/1
  PdTelemetry/2(telQ) -> p1c_telQ/1
  Timing Adjust/4(p1c_armed) -> PdTelemetry/11(armed)
  Timing Adjust/3(SyncPulse) -> Delay4/1, PdTelemetry/10(sync)  "synchronizedPulse"
  P1cSplit/2 -> P1cDSi2/1
  P1cSplit/1 -> P1cDSi1/1
  Delay11/1 -> Timing Adjust/1(timingOffset)
  Peak Search/1(timingOffset) -> P1cToffSi/1, Delay11/1
  Correlator/1(dataOut) -> No HDL/1(In1), Relational Operator/1, Peak Search/1(corr)
  PdPopIndex/1(pop) -> FIFO/3(pop), Delay14/1
  validIn/1 -> Delay2/1
  Delay8/1 -> PdPopIndex/1(delay8Out), FIFO/2(push)
  Delay5/1 -> validOut/1
  Delay13/1 -> Timing Adjust/3(dataIn)
  Relational Operator/1 -> Peak Search/2(thresholdExceeded), PdTelemetry/4(thrEx)
  Delay/1 -> Delay6/1
  Delay2/1 -> Delay7/1, Correlator/2(validIn), PdTelemetry/1(validIn)
  Delay3/1 -> dataOut/1
  FIFO/3(validPop) -> Terminator1/1, PdTelemetry/15(vPop)
  P1cTlongSi/1 -> PdTelemetry/16(tRefLong)
  Peak Search/4(p1c_tref) -> P1cTrefSi/1
  Timing Adjust/1(dataOut) -> Delay3/1  "synchronizedData"
  Delay14/1 -> Timing Adjust/4(validIn)
  Correlator/3(validOut) -> No HDL/Enable, Peak Search/3(validIn)
  dataIn/1 -> Delay1/1
  Timing Adjust/2(validOut) -> Delay5/1  "synchronizedValid"
  Delay12/1 -> Timing Adjust/2(timingOffsetValid)
  Delay1/1 -> Delay/1, Correlator/1(dataIn), P1cSplit/1
  Peak Search/2(done) -> Logical Operator/1, PdTelemetry/7(done)  "done"
  Correlator/2(threshold) -> Relational Operator/2, No HDL/2(In2)
  Constant/1 -> FIFO/4(reset)
  Logical Operator/1 -> Delay12/1
  Peak Search/6(p1c_runmax) -> fs_runmax/1, P1cRmaxSi/1
  Peak Search/5(p1c_treflong) -> P1cTlongSi/1
  Peak Search/8(p1c_heldts) -> P1cHeldSi/1
  FIFO/1(out) -> Delay13/1
  Peak Search/3(success) -> Logical Operator/2, PdTelemetry/9(succ)  "success"
  Delay6/1 -> FIFO/1(in)
  P1cTrefSi/1 -> PdTelemetry/5(tRef)
  Peak Search/7(p1c_newpk) -> PdTelemetry/8(newPk)
  Delay7/1 -> Delay8/1
  P1cToffSi/1 -> PdTelemetry/6(tOff)
  FIFO/2(numEntries) -> PdPopEntSi/1, Terminator/1, P1cEntSi/1
  P1cDSi2/1 -> PdTelemetry/3(dQ)
  PdPopEntSi/1 -> PdPopIndex/2(numEntries)

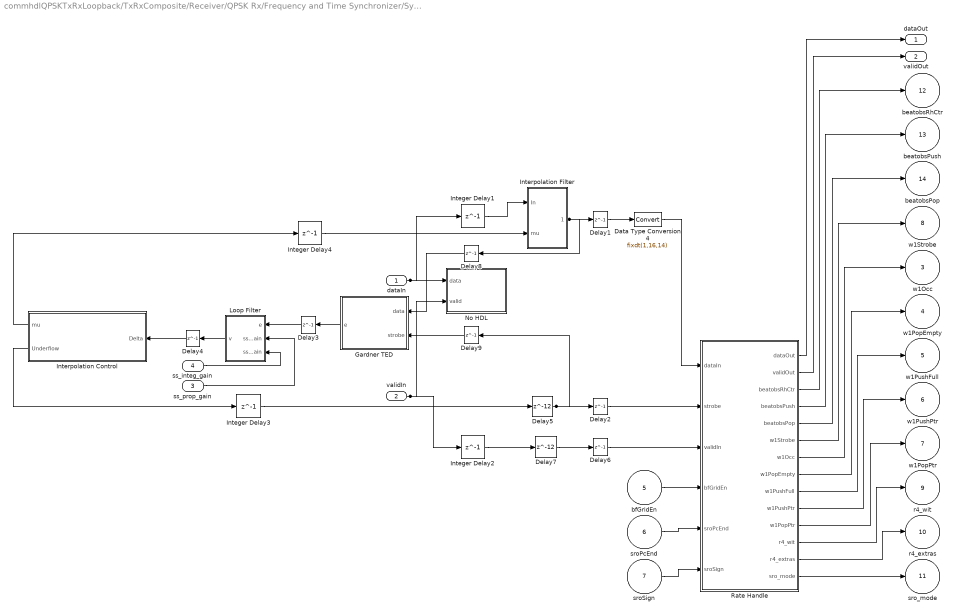
== system commhdlQPSKTxRxLoopback/TxRxComposite/Receiver/QPSK Rx/Frequency and Time Synchronizer/Symbol Synchronizer ==
  dataIn : Inport
  validIn : Inport  Port=2
  ss_prop_gain : Inport  Port=3  OutDataTypeStr=uint32  SampleTime=1/(Rsym*SamplesPerSymbol)
  ss_integ_gain : Inport  Port=4  OutDataTypeStr=uint32  SampleTime=1/(Rsym*SamplesPerSymbol)
  bfGridEn : Inport  Port=5  OutDataTypeStr=boolean
  sroPcEnd : Inport  Port=6  OutDataTypeStr=boolean
  sroSign : Inport  Port=7  OutDataTypeStr=boolean
  Data Type Conversion4 : DataTypeConversion  OutDataTypeStr=fixdt(1,16,14)  SaturateOnIntegerOverflow=off  RndMeth=Floor
  Delay{1..4,6,8..9} (7 alike) : Delay  DelayLength=1
  Delay5 : Delay  DelayLength=12
  Delay7 : Delay  DelayLength=12
  Gardner TED : Subsystem
  Integer Delay{1..4} (4 alike) : Delay  DelayLength=1
  Interpolation Control : MATLAB Function
  Interpolation Filter : Subsystem
  Loop Filter : Subsystem
  No HDL : Subsystem
  Rate Handle : Subsystem  Description=Rate Handle: turns the Symbol Synchronizer's strobe-timed (irregular) symbol output into a regular 1-in-4 symbol stream through a small FIFO (push on strobe, pop on the mod-4 grid). Overlays added the bfGridEn pacer (fixctl bit 2), the beatobs/W1 witness taps, and RxSteer pop steering (fixctl bit 5 = sroSign). See the notes inside the subsystem.
  dataOut : Outport
  validOut : Outport  Port=2
  w1Occ : Outport  Port=3
  w1PopEmpty : Outport  Port=4
  w1PushFull : Outport  Port=5
  w1PushPtr : Outport  Port=6
  w1PopPtr : Outport  Port=7
  w1Strobe : Outport  Port=8
  r4_wit : Outport  Port=9
  r4_extras : Outport  Port=10
  sro_mode : Outport  Port=11
  beatobsRhCtr : Outport  Port=12
  beatobsPush : Outport  Port=13
  beatobsPop : Outport  Port=14
  wires:
  Rate Handle/14(sro_mode) -> sro_mode/1
  Rate Handle/13(r4_extras) -> r4_extras/1
  Rate Handle/9(w1PushFull) -> w1PushFull/1
  Rate Handle/8(w1PopEmpty) -> w1PopEmpty/1
  Rate Handle/6(w1Strobe) -> w1Strobe/1
  Rate Handle/4(beatobsPush) -> beatobsPush/1
  dataIn/1 -> No HDL/1(data), Integer Delay1/1
  Gardner TED/1(e) -> Delay3/1
  Data Type Conversion4/1 -> Rate Handle/1(dataIn)
  sroSign/1 -> Rate Handle/6(sroSign)
  Rate Handle/11(w1PopPtr) -> w1PopPtr/1
  validIn/1 -> No HDL/2(valid), Integer Delay2/1
  ss_prop_gain/1 -> Loop Filter/2(ss_prop_gain)
  Integer Delay3/1 -> Delay5/1
  Delay3/1 -> Loop Filter/1(e)
  Loop Filter/1(v) -> Delay4/1
  Interpolation Control/1(mu) -> Integer Delay4/1
  Integer Delay4/1 -> Interpolation Filter/2(mu)
  sroPcEnd/1 -> Rate Handle/5(sroPcEnd)
  ss_integ_gain/1 -> Loop Filter/3(ss_integ_gain)
  Rate Handle/10(w1PushPtr) -> w1PushPtr/1
  Delay2/1 -> Rate Handle/2(strobe)
  Rate Handle/5(beatobsPop) -> beatobsPop/1
  Delay4/1 -> Interpolation Control/1(Delta)
  Interpolation Control/2(Underflow) -> Integer Delay3/1
  Delay5/1 -> Delay2/1, Delay9/1
  Rate Handle/12(r4_wit) -> r4_wit/1
  Delay8/1 -> Gardner TED/1(data)
  Delay9/1 -> Gardner TED/2(strobe)
  Delay1/1 -> Data Type Conversion4/1
  Integer Delay1/1 -> Interpolation Filter/1(In)
  Rate Handle/7(w1Occ) -> w1Occ/1
  Interpolation Filter/1(interpolant) -> Delay1/1, Delay8/1
  Delay6/1 -> Rate Handle/3(validIn)
  Delay7/1 -> Delay6/1
  bfGridEn/1 -> Rate Handle/4(bfGridEn)
  Integer Delay2/1 -> Delay7/1
  Rate Handle/1(dataOut) -> dataOut/1
  Rate Handle/2(validOut) -> validOut/1
  Rate Handle/3(beatobsRhCtr) -> beatobsRhCtr/1

== system commhdlQPSKTxRxLoopback/TxRxComposite/Receiver/QPSK Rx/QPSK Demodulator/Serializer ==
  u : Inport
  In2 : Inport  Port=2
  bfAnchor : Inport  Port=3  OutDataTypeStr=boolean
  BfSerMux : MATLAB Function  TreatAsAtomicUnit=on
  Delay1 : Delay  DelayLength=1
  Delay4 : Delay  DelayLength=1
  Demux : Demux  Outputs=2
  HDL Counter : hdlsllib/Sources/HDL Counter  CountType=Count limited  CountInit=0  CountStep=1  CountMax=1  CountFromType=Initial value  CountFrom=0  CountResetPort=off  CountLoadPort=off  CountEnbPort=on  CountDirPort=off  CountHitOutputPort=off  CountDataType=Unsigned  CountWordLen=1  CountFracLen=0  CountSampTime=1
  Logical Operator : Logic  Operator=OR  AllPortsSameDT=off  OutDataTypeStr=boolean
  Multiport Switch : MultiPortSwitch  DataPortOrder=Zero-based contiguous  Inputs=2  zeroidx=on  SaturateOnIntegerOverflow=off  InputSameDT=off
  Unit Delay Enabled Synchronous : hdlsllib/Discrete/Unit Delay Enabled Synchronous  InitialCondition=0.0  SampleTime=-1
  Out1 : Outport
  Out2 : Outport  Port=2
  wires:
  Demux/2 -> Multiport Switch/3
  BfSerMux/1(y) -> Multiport Switch/1
  Demux/1 -> Multiport Switch/2
  bfAnchor/1 -> BfSerMux/2(anchor)
  Logical Operator/1 -> Out2/1, HDL Counter/1
  Multiport Switch/1 -> Out1/1
  HDL Counter/1 -> BfSerMux/1(c)
  Delay4/1 -> Logical Operator/2
  Unit Delay Enabled Synchronous/1 -> Demux/1
  Delay1/1 -> Delay4/1, Logical Operator/1
  u/1 -> Unit Delay Enabled Synchronous/1
  In2/1 -> Unit Delay Enabled Synchronous/2, Delay1/1

== system commhdlQPSKTxRxLoopback/TxRxComposite/Transmitter/QPSK Tx/Bit Packetizer/Data Bits FIFO ==
  data : Inport
  push : Inport  Port=2
  Compare To Constant : simulink/Logic and Bit Operations/Compare To Constant  relop=>=  const=length(Preamble)  OutDataTypeStr=boolean
  Compare To Constant1 : simulink/Logic and Bit Operations/Compare To Constant  relop===  const=0  OutDataTypeStr=boolean
  Compare To Constant2 : simulink/Logic and Bit Operations/Compare To Constant  relop=~=  const=0  OutDataTypeStr=boolean
  Compare To Constant3 : simulink/Logic and Bit Operations/Compare To Constant  relop===  const=0  OutDataTypeStr=boolean
  Compare To Constant4 : simulink/Logic and Bit Operations/Compare To Constant  relop===  const=bitsPerPacket - 1  OutDataTypeStr=boolean
  Compare To Constant5 : hdlsllib/Logic and Bit Operations/Compare To Constant  relop=>=  const=Config.SamplesPerSymbol/2 -1  OutDataTypeStr=boolean
  Constant : Constant  Value=true  SampleTime=1/(Rsym*SamplesPerSymbol)
  Delay{1..7} (7 alike) : Delay  DelayLength=1
  HDL Counter : hdlsllib/Sources/HDL Counter  CountType=Count limited  CountInit=0  CountStep=1  CountMax=dataBitsPerPacket*2 - 1  CountFromType=Initial value  CountFrom=0  CountResetPort=off  CountLoadPort=off  CountEnbPort=on  CountDirPort=off  CountHitOutputPort=off  CountDataType=Unsigned  CountWordLen=nextpow2(dataBitsPerPacket*2 - 1)  CountFracLen=0  CountSampTime=1
  HDL Counter1 : hdlsllib/Sources/HDL Counter  CountType=Count limited  CountInit=0  CountStep=1  CountMax=dataBitsPerPacket*2 - 1  CountFromType=Initial value  CountFrom=0  CountResetPort=off  CountLoadPort=off  CountEnbPort=on  CountDirPort=off  CountHitOutputPort=off  CountDataType=Unsigned  CountWordLen=nextpow2(dataBitsPerPacket*2 - 1)  CountFracLen=0  CountSampTime=1
  HDL Counter2 : hdlsllib/Sources/HDL Counter  CountType=Count limited  CountInit=0  CountStep=1  CountMax=bitsPerPacket - 1  CountFromType=Initial value  CountFrom=0  CountResetPort=off  CountLoadPort=off  CountEnbPort=on  CountDirPort=off  CountHitOutputPort=off  CountDataType=Unsigned  CountWordLen=nextpow2(bitsPerPacket)  CountFracLen=0  CountSampTime=1
  HDL Counter3 : hdlsllib/Sources/HDL Counter  CountType=Count limited  CountInit=0  CountStep=1  CountMax=max(1, Config.SamplesPerSymbol/2 -1)  CountFromType=Initial value  CountFrom=0  CountResetPort=off  CountLoadPort=off  CountEnbPort=on  CountDirPort=off  CountHitOutputPort=off  CountDataType=Unsigned  CountWordLen=max(1, nextpow2(Config.SamplesPerSymbol/2))  CountFracLen=0  CountSampTime=1
  Logical Operator : Logic  Inputs=3  AllPortsSameDT=off  OutDataTypeStr=boolean
  Logical Operator1 : Logic  Inputs=3  AllPortsSameDT=off  OutDataTypeStr=boolean
  MATLAB Function1 : MATLAB Function  TreatAsAtomicUnit=on
  No HDL : Subsystem
  RAM Frame Status Indicator : MATLAB Function  TreatAsAtomicUnit=on
  Simple Dual Port RAM : hdlsllib/HDL RAMs/Simple Dual Port RAM  ram_size=nextpow2(dataBitsPerPacket*2 - 1)
  TxF1BoundaryGuard : Logic  AllPortsSameDT=off  OutDataTypeStr=boolean
  Unit Delay Enabled Resettable Synchronous : hdlsllib/Discrete/Unit Delay Enabled Resettable Synchronous  InitialCondition=0.0  SampleTime=-1
  dataOut : Outport
  activeFrame : Outport  Port=2
  sampleCount : Outport  Port=3
  sampleCountValid : Outport  Port=4
  fullRAM : Outport  Port=5
  wires:
  MATLAB Function1/1(full) -> Delay7/1
  HDL Counter1/1 -> Simple Dual Port RAM/4
  HDL Counter/1 -> Simple Dual Port RAM/2
  Delay7/1 -> fullRAM/1
  data/1 -> Simple Dual Port RAM/1
  RAM Frame Status Indicator/1(out) -> Delay3/1
  Logical Operator1/1 -> activeFrame/1
  push/1 -> MATLAB Function1/1(wr), Simple Dual Port RAM/3, HDL Counter/1, No HDL/1(push), RAM Frame Status Indicator/1(push)
  Delay6/1 -> Logical Operator1/3, sampleCountValid/1
  Logical Operator/1 -> HDL Counter1/1, RAM Frame Status Indicator/2(pop), MATLAB Function1/2(rd), No HDL/2(pop)
  Unit Delay Enabled Resettable Synchronous/1 -> Logical Operator/1
  Compare To Constant4/1 -> Logical Operator1/2
  Delay3/1 -> Compare To Constant2/1, Compare To Constant1/1
  Constant/1 -> HDL Counter3/1
  Compare To Constant1/1 -> TxF1BoundaryGuard/1
  Delay2/1 -> Delay5/1
  Compare To Constant/1 -> Delay1/1
  Compare To Constant5/1 -> HDL Counter2/1, Delay4/1
  Delay5/1 -> Compare To Constant4/1, sampleCount/1
  HDL Counter3/1 -> Compare To Constant5/1
  HDL Counter2/1 -> Compare To Constant/1, Delay2/1, Compare To Constant3/1
  Delay1/1 -> Logical Operator/2
  Compare To Constant2/1 -> Unit Delay Enabled Resettable Synchronous/1, Logical Operator1/1
  Simple Dual Port RAM/1 -> dataOut/1
  Delay4/1 -> Delay6/1, Logical Operator/3
  Compare To Constant3/1 -> TxF1BoundaryGuard/2, Unit Delay Enabled Resettable Synchronous/2
  TxF1BoundaryGuard/1 -> Unit Delay Enabled Resettable Synchronous/3

== system commhdlQPSKTxRxLoopback/TxRxComposite/Transmitter/QPSK Tx/Bit Packetizer/Preamble Bits Generator ==
  activeFrame : Inport
  sampleCount : Inport  Port=2
  sampleCountValid : Inport  Port=3
  Compare To Constant2 : hdlsllib/Logic and Bit Operations/Compare To Constant  relop===  const=bitsPerPacket - 1  OutDataTypeStr=boolean
  Logical Operator3 : Logic  AllPortsSameDT=off  OutDataTypeStr=boolean
  Preamble Bits Store : Subsystem
  Unit Delay Enabled Synchronous : hdlsllib/Discrete/Unit Delay Enabled Synchronous  InitialCondition=0.0  SampleTime=-1
  preambleBits : Outport
  wires:
  Unit Delay Enabled Synchronous/1 -> Preamble Bits Store/1(actualPreamble)
  Logical Operator3/1 -> Unit Delay Enabled Synchronous/2
  activeFrame/1 -> Unit Delay Enabled Synchronous/1
  sampleCountValid/1 -> Logical Operator3/2
  Preamble Bits Store/1(preamble) -> preambleBits/1
  Compare To Constant2/1 -> Logical Operator3/1
  sampleCount/1 -> Compare To Constant2/1, Preamble Bits Store/2(sampleCount)

== system commhdlQPSKTxRxLoopback/Receiver/QPSK Rx/Frequency and Time Synchronizer/Coarse Frequency Compensator/Coarse Frequency Estimator/Extract Frequency ==
  datain : Inport
  validIn : Inport  Port=2
  Complex to Magnitude-Angle HDL Optimized : dsphdlmathfun2/Complex to Magnitude-Angle  NumIterationsSource=Auto  NumIterations=10  OutputFormat=Angle  AngleFormat=Normalized  ScaleOutput=on  ScalingMethod=Shift-Add  SimulateUsing=Code generation
  Delay{1..4} (4 alike) : Delay  DelayLength=1
  Gain : Gain  Gain=1/2  ParamDataTypeStr=fixdt(0,1,1)  OutDataTypeStr=Inherit: Same as input
  Unit Delay Enabled Synchronous : hdlsllib/Discrete/Unit Delay Enabled Synchronous  InitialCondition=0.0  SampleTime=-1
  normFreqOut : Outport
  wires:
  Unit Delay Enabled Synchronous/1 -> Delay2/1
  Complex to Magnitude-Angle HDL Optimized/2 -> Unit Delay Enabled Synchronous/2
  datain/1 -> Delay1/1
  Gain/1 -> Delay3/1
  Delay1/1 -> Complex to Magnitude-Angle HDL Optimized/1
  Delay2/1 -> Gain/1
  Delay3/1 -> normFreqOut/1
  validIn/1 -> Delay4/1
  Delay4/1 -> Complex to Magnitude-Angle HDL Optimized/2
  Complex to Magnitude-Angle HDL Optimized/1 -> Unit Delay Enabled Synchronous/1

== system commhdlQPSKTxRxLoopback/Receiver/QPSK Rx/Frequency and Time Synchronizer/Coarse Frequency Compensator/Coarse Frequency Estimator/Integrator ==
  note: store the value in the Reg before reset
  dataIn : Inport
  validIn : Inport  Port=2
  Add1 : Sum  Inputs=|++  OutDataTypeStr=Inherit: Same as first input
  Delay : Delay  DelayLength=1
  Delay1 : Delay  DelayLength=1
  Delay2 : Delay  DelayLength=1
  Integ Reg : hdlsllib/Discrete/Unit Delay Enabled Resettable Synchronous  InitialCondition=0.0  SampleTime=-1
  Reset Generator : Subsystem
  Store Reg : hdlsllib/Discrete/Unit Delay Enabled Synchronous  InitialCondition=0.0  SampleTime=-1
  IntegOut : Outport
  IntegValid : Outport  Port=2
  wires:
  Add1/1 -> Integ Reg/1
  Integ Reg/1 -> Store Reg/1, Add1/2
  validIn/1 -> Delay2/1, Reset Generator/1(validIn)
  dataIn/1 -> Delay1/1
  Delay1/1 -> Add1/1
  Delay/1 -> IntegValid/1
  Store Reg/1 -> IntegOut/1
  Reset Generator/1(reset) -> Delay/1, Store Reg/2, Integ Reg/3
  Delay2/1 -> Integ Reg/2
